simulink model "Analog_lector"  (R2026a)
settings: Solver=FixedStepAuto  StopTime=inf  FixedStep=0.1  EnableMultiTasking=on
libraries: arduinolib x1, simulink_extras x1
settings Model: SILPILModeSetting=veronly  ExtModeTrigDuration=2  Creator=Resen  LastModifiedBy=Resen
settings HardwareCC: ProdBitPerInt=16.0  ProdBitPerPointer=16.0  ProdBitPerSizeT=16.0  ProdBitPerPtrDiffT=16.0  ProdWordSize=8.0  ProdHWDeviceType=Atmel->AVR  UseEmbeddedCoderFeatures=off  UseSimulinkCoderFeatures=off
settings RTWCC: SystemTargetFile=ert.tlc  HardwareBoard=Arduino Uno  TLCOptions=-aInlineSetEventsForThisBaseRateFcn=TLC_FALSE -aSuppressMultiTaskScheduler=TLC_FALSE -aRateBasedStepFcn=1  Toolchain=Arduino AVR  BuildConfiguration=Faster Runs  Description=Embedded Coder
settings ERTTargetCC: ExtModeTransport=3.0  ExtModeAutomaticAllocSize=off  ExtModeStaticAllocSize=250.0  SupportContinuousTime=on  SupportNonInlinedSFcns=on  SupportVariableSizeSignals=on

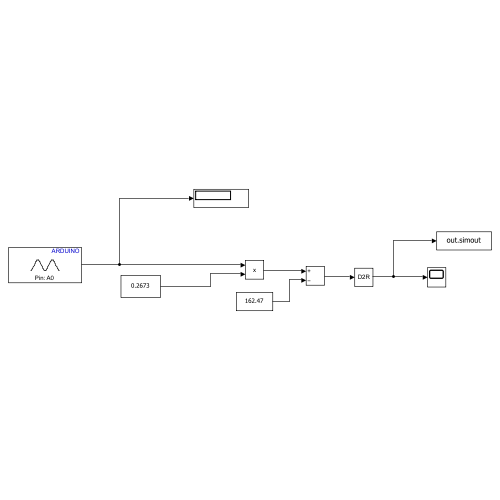
[thumbnail: Simulink's stored preview of the top-level diagram]
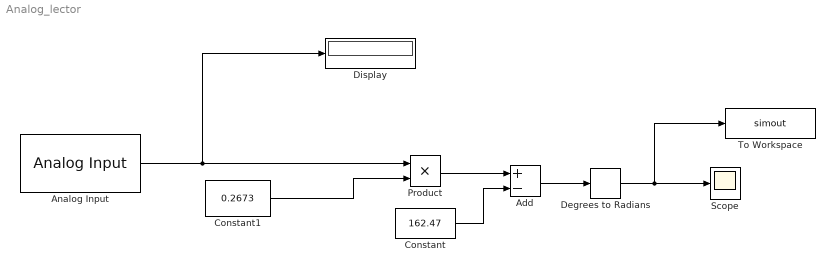
== system Analog_lector ==
  Add : Sum  Inputs=+-
  Analog Input : arduinolib/Analog Input  pinNumber=0  ReadResultsOnly=off  ConversionTriggerSource=Software  ExternalTriggerType=uint32( 0 )  OutputDataType=uint16  EnableConversionCompleteNotify=off  EnableOuputStatus=off  SampleTime=-1  blockPlatform=arduino
      settings: LibrarySourceBlock=gizmoLibrary/Arduino Utilities/Analog Input
  Constant : Constant  Value=162.47
  Constant1 : Constant  Value=0.2673
  Degrees to Radians : simulink_extras/Transformations/Degrees to Radians
  Display : Display
  Product : Product
  Scope : Scope
      settings: TimeSpan=100  ActiveDisplayYMinimum=-1.6  ActiveDisplayYMaximum=1.6
  To Workspace : ToWorkspace  VariableName=simout  SampleTime=-1
      settings: Save2DSignal=2-D array (concatenate along first dimension)
  wires:
  Analog Input/1 -> Display/1, Product/1
  Constant1/1 -> Product/2
  Product/1 -> Add/1
  Constant/1 -> Add/2
  Add/1 -> Degrees to Radians/1
  Degrees to Radians/1 -> To Workspace/1, Scope/1
